simulink library "Steer_Rack_WheelDrivenRack"  (R2025a)
settings: Solver=VariableStepAuto  StartTime=0.0  StopTime=10.0  RelTol=1e-3
undefined symbols (not defined in the file): Steer, Vehicle, Visual, X, Y, Z
libraries: sm_lib x30, nesl_utility x4, Vehicle_Inputs x1, Driver_Systems x1, SteeringWheel x1
Description:
  | Component of Simscape Vehicle Templates Library
  | 
  | Copyright 2018-2026 The MathWorks, Inc.
settings Model: Creator=smiller  LastModifiedBy=smiller
settings OptimizationCC: ReuseModelBlockBuffer=off
settings ModelReferenceCC: EnableRefExpFcnMdlSchedulingChecks=on
settings RTWCC: GPUComputeCapability=3.5

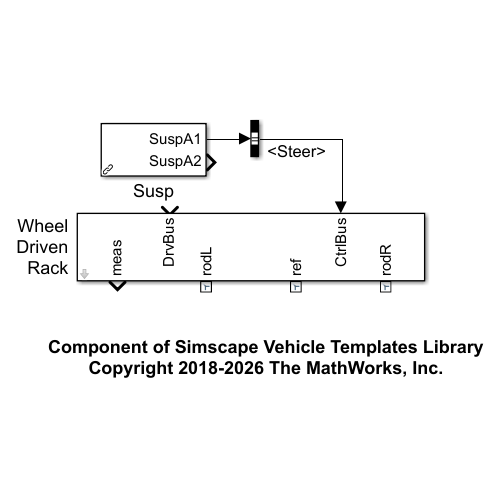
[thumbnail: Simulink's stored preview of the top-level diagram]
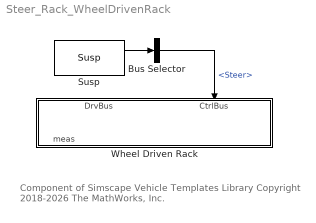
== system Steer_Rack_WheelDrivenRack ==
  note: Component of Simscape Vehicle Templates Library
      | Copyright 2018-2026 The MathWorks, Inc.
  Bus Selector : BusSelector  OutputSignals=Steer
  Susp : Vehicle_Inputs/Control Bus/Susp  SystemSampleTime=-1  VariantActivationTime=update diagram  EmptyChoice=off  PassThrough=off  PassThroughVariantControl=(default)  EmptyChoiceVariantControl=(default)  AllowFlexibleInterface=on  Latency=0  AutoFrameSizeCalculation=off
  Wheel Driven Rack : Subsystem  Tag=PublishSubsystem  VariantControl=Rack  mask(Steering System with Wheel Actuation){hp_wheel=Vehicle.Chassis.SuspF.Steer.Wheel.sMount.Value, wheel_axis_incl=Vehicle.Chassis.SuspF.Steer.Wheel.aAxis.Value, hp_mt_rack=Vehicle.Chassis.SuspF.Steer.Rack.sMount.Value, hp_out_rack=Vehicle.Chassis.SuspF.Steer.Rack.sOutboard.Value, hp_pinion=Vehicle.Chassis.SuspF.Steer.Pinion.sMount.Value, Wheel=Steer.Wheel, len_sha_u=Vehicle.Chassis.SuspF.Steer.Shaft_Upper.xLength.Value, sha_u_mass=Vehicle.Chassis.SuspF.Steer.Shaft_Upper.m.Value, sha_i_mass=Vehicle.Chassis.SuspF.Steer.Shaft_Intermediate.m.Value, len_sha_l=Vehicle.Chassis.SuspF.Steer.Shaft_Lower.xLength.Value, sha_l_mass=Vehicle.Chassis.SuspF.Steer.Shaft_Lower.m.Value, rad_pinion=Vehicle.Chassis.SuspF.Steer.Pinion.xRad.Value, pinion_mass=Vehicle.Chassis.SuspF.Steer.Pinion.m.Value, rack_mass=Vehicle.Chassis.SuspF.Steer.Rack.m.Value, whl2steer_filter=1/Vehicle.Chassis.SuspF.Steer.Rack.fActuatorCutoff.Value, clr_rack=Visual.SteeringRack.clr, opc_rack=Visual.part.opc, radius_rack=Visual.SteeringRack.rad, clr_shaft=Visual.SteeringShafts.clr, opc_shaft=Visual.part.opc, size_shaft=Visual.SteeringShafts.rad, clr_pinion=Visual.SteeringPinion.clr, opc_pinion=Visual.part.opc, len_pinion=Visual.SteeringPinion.len, clr_connhp=Visual.hp.clr, opc_connhp=Visual.hp.opc, size_connhp=Visual.hp.rad, clr_wheel=Visual.SteeringWheel.clr, opc_wheel=Visual.part.opc, DriverHuman=Steer.DriverHuman}
      mask prompts: hp_wheel "HP Wheel [xyz] (m)"; wheel_axis_incl "Wheel Axis Angle (rad)"; hp_mt_rack "HP Rack Mount [xyz] (m)"; hp_out_rack "HP Track Rod Inboard [xyz] (m)"; hp_pinion "HP Pinion [xyz] (m)"; whl2steer_filter "Steer Motion Filter (sec)"; DriverHuman "Driver Human (structure)"
      mask help: Actuation is applied to steering wheel and transmitted to rack via shafts in steering column. Assumes constant gear ratio between pinion and rack.
      mask init:
      | % Calculate inclination of pinion gear about rack travel axis
      | pinion_incl = atan2(hp_mt_rack(1)-hp_pinion(1),hp_mt_rack(3)-hp_pinion(3));
      | 
      | % Calculate endpoints of lower column and upper column
      | hp_col_lower = hp_pinion + [-len_sha_l*cos(pinion_incl) 0 len_sha_l*sin(pinion_incl)];
      | hp_col_upper = hp_wheel  + [+len_sha_u*cos(wheel_axis_incl)  0 -len_sha_u*sin(wheel_axis_incl)];
      | 
      | % Calculate length of intermediate shaft
      | len_sha_int  = norm(hp_col_upper-hp_col_lower);
      mask TypeOptions hp_wheel:
      | Ref to Wheel/Transform
      | HP Wheel/TranslationCartesianOffset
      mask TypeOptions hp_mt_rack:
      | Ref to Rack/Transform
      | HP Rack/TranslationCartesianOffset
      mask TypeOptions hp_out_rack: Rack/hp_out
      mask TypeOptions rack_mass: Rack/rack_mass
      mask TypeOptions whl2steer_filter: Physical Signal/InputFilterTimeConstant
      mask TypeOptions clr_rack: Rack/clr_rack
      mask TypeOptions opc_rack: Rack/opc_rack
      mask TypeOptions radius_rack: Rack/radius_rack
      mask TypeOptions clr_shaft:
      | Shaft
      | Steering/Shaft/GraphicDiffuseColor | Shaft
      | Lower/Shaft/GraphicDiffuseColor | Shaft
      | Intermediate/Shaft/GraphicDiffuseColor
      mask TypeOptions opc_shaft:
      | Shaft
      | Steering/Shaft/GraphicOpacity | Shaft
      | Lower/Shaft/GraphicOpacity | Shaft
      | Intermediate/Shaft/GraphicOpacity
      mask TypeOptions size_shaft:
      | Shaft
      | Steering/Shaft/CylinderRadius | Shaft
      | Lower/Shaft/CylinderRadius | Shaft
      | Intermediate/Shaft/CylinderRadius
      mask TypeOptions clr_pinion: Pinion/Pinion/GraphicDiffuseColor
      mask TypeOptions opc_pinion: Pinion/Pinion/GraphicOpacity
      mask TypeOptions len_pinion: Pinion/Pinion/CylinderLength
      mask TypeOptions clr_connhp:
      | Ref to Rack/Vis
      | Rack
      | Housing/GraphicDiffuseColor | HPs/HP Lower Col/GraphicDiffuseColor | HPs/HP Pinion/GraphicDiffuseColor | HPs/HP Upper Col/GraphicDiffuseColor
      mask TypeOptions opc_connhp:
      | Ref to Rack/Vis
      | Rack
      | Housing/GraphicOpacity | HPs/HP Lower Col/GraphicOpacity | HPs/HP Pinion/GraphicOpacity | HPs/HP Upper Col/GraphicOpacity
      mask TypeOptions size_connhp:
      | Ref to Rack/Vis
      | Rack
      | Housing/SphereRadius | HPs/HP Lower Col/SphereRadius | HPs/HP Pinion/SphereRadius | HPs/HP Upper Col/SphereRadius
      mask TypeOptions clr_wheel: Wheel/clr_wheel
      mask TypeOptions opc_wheel: Wheel/opc_wheel
      mask DialogControl cont_steer Prompt: Steer
      mask DialogControl grp_strparts Prompt: Parts
      mask DialogControl text_strparts_len Prompt: Length/Radius (m)
      mask DialogControl text_strparts_mass Prompt: Mass (kg)
      mask DialogControl text_strparts_wheel Prompt: Wheel
      mask DialogControl text_strparts_wheel_m Prompt: <CAD file>
      mask DialogControl text_strparts_sha_u Prompt: Upper Shaft
      mask DialogControl text_strparts_sha_i Prompt: Intermediate Shaft
      mask DialogControl text_strparts_sha_i_len Prompt: <length upper, lower>
      mask DialogControl text_strparts_sha_len Prompt: Lower Shaft
      mask DialogControl text_strparts_pinion Prompt: Pinion
      mask DialogControl text_strparts_rack Prompt: Rack
      mask DialogControl text_strparts_rack_len Prompt: <HP Rod Inboard>
      mask DialogControl grp_steering Prompt: Steering Input
      mask DialogControl cont_vis_steer Prompt: Visualization
      mask DialogControl text_steer_vis_clr Prompt: Color [RGB]
      mask DialogControl text_steer_vis_opc Prompt: Opac. (0-1)
      mask DialogControl text_steer_vis_size Prompt: Size (m)
      mask DialogControl text_steer_vis_rack Prompt: Rack
      mask DialogControl text_steer_vis_shafts Prompt: Shafts
      mask DialogControl text_steer_vis_pinion Prompt: Pinion
      mask DialogControl text_steer_vis_connhp Prompt: Connections, HP
      mask DialogControl text_steer_vis_wheel Prompt: Wheel
      mask DialogControl text_steer_size_wheel Prompt: <CAD File>
      mask DialogControl cont_driver_human Prompt: Driver Human
  wires:
  Bus Selector/1 -> Wheel Driven Rack/2(CtrlBus)  "<Steer>"
  Susp/1 -> Bus Selector/1

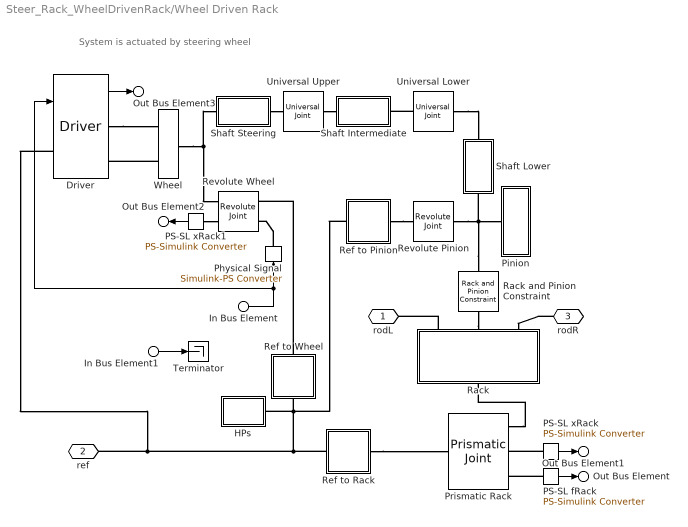
== system Steer_Rack_WheelDrivenRack/Wheel Driven Rack ==
  note: System is actuated by
      | steering wheel
  In Bus Element1 : Inport  PortName=DrvBus  Element=aSteerWheel
  In Bus Element : Inport  Port=2  PortName=CtrlBus  Element=aSteerWheel
  Driver : Driver_Systems/Driver  LabelModeActiveChoice=Human  DriverHuman=DriverHuman  VariantLabel=DriverHuman.class.Value
      settings: AttributesFormatString=%<LabelModeActiveChoice>
  HPs : Subsystem
  PS-SL fRack : nesl_utility/PS-Simulink Converter  PhysicalDomain=network_engine_domain  SubClassName=ps_output  LeftPortType=input  RightPortType=output  PseudoPeriodic=off  Frequencies=[]  VectorFormat=1-D array  Unit=1  AffineConversion=off
  PS-SL xRack : nesl_utility/PS-Simulink Converter  PhysicalDomain=network_engine_domain  SubClassName=ps_output  LeftPortType=input  RightPortType=output  PseudoPeriodic=off  Frequencies=[]  VectorFormat=1-D array  Unit=1  AffineConversion=off
  PS-SL xRack1 : nesl_utility/PS-Simulink Converter  PhysicalDomain=network_engine_domain  SubClassName=ps_output  LeftPortType=input  RightPortType=output  PseudoPeriodic=off  Frequencies=[]  VectorFormat=1-D array  Unit=rad  AffineConversion=off
  Physical Signal : nesl_utility/Simulink-PS Converter  PhysicalDomain=network_engine_domain  SubClassName=ps_input  LeftPortType=input  RightPortType=output  PseudoPeriodic=off  Frequencies=[]  NoiseDistribution=none  NoiseParameters=[]  Unit=rad  AffineConversion=off  FilteringAndDerivatives=filter  SimscapeFilterOrder=2  InputFilterTimeConstant=whl2steer_filter  UdotUserProvided=0
      settings: AttributesFormatString=|
      | Filter Time Constant
      | %<InputFilterTimeConstant> sec
  Pinion : Subsystem
  Prismatic Rack : sm_lib/Joints/Prismatic Joint  JointMode=Normal  CompositeWrenchDir=FollowerOnBase  CompositeWrenchFrame=BaseFrame  SenseConstraintForce=off  SenseConstraintTorque=off  SenseTotalForce=off  SenseTotalTorque=off  PositionTargetSpecify=on  PositionTargetPriority=High  PositionTargetValue=0  PositionTargetValueUnits=m  VelocityTargetSpecify=off  VelocityTargetPriority=High  VelocityTargetValue=0  VelocityTargetValueUnits=m/s  EquilibriumPosition=0  EquilibriumPositionUnits=m  SpringStiffness=0  SpringStiffnessUnits=N/m  DampingCoefficient=1e5*0  DampingCoefficientUnits=N/(m/s)  LowerLimitSpecify=off  LowerLimitBound=-1  LowerLimitBoundUnits=m  LowerLimitStiffness=1e6  LowerLimitStiffnessUnits=N/m  LowerLimitDamping=1e3  LowerLimitDampingUnits=N/(m/s)  LowerLimitTransitionRegionWidth=1e-4  LowerLimitTransitionRegionWidthUnits=m  UpperLimitSpecify=off  UpperLimitBound=1  UpperLimitBoundUnits=m  UpperLimitStiffness=1e6  UpperLimitStiffnessUnits=N/m  UpperLimitDamping=1e3  UpperLimitDampingUnits=N/(m/s)  UpperLimitTransitionRegionWidth=1e-4  UpperLimitTransitionRegionWidthUnits=m  TorqueActuationMode=NoTorque  MotionActuationMode=ComputedMotion  SensePosition=on  SenseVelocity=off  SenseAcceleration=off  SenseTorqueForce=on  SenseLowerLimitTorqueForce=off  SenseUpperLimitTorqueForce=off
  Rack : Subsystem  mask{hp_out=hp_out_rack, rack_mass=rack_mass, clr_rack=clr_rack, opc_rack=opc_rack, radius_rack=radius_rack}
      mask prompts: hp_out "HP Track Rod Inboard [xyz] (m)"; rack_mass "Mass (kg)"
      mask init:
      | rack_length = norm(hp_out-hp_out.*[1 -1 1]);
      mask TypeOptions rack_mass: Rack/Mass
      mask TypeOptions clr_rack: Rack/GraphicDiffuseColor
      mask TypeOptions opc_rack: Rack/GraphicOpacity
      mask TypeOptions radius_rack: Rack/CylinderRadius
      mask DialogControl cont_rack Prompt: Rack
      mask DialogControl text_rack_clr Prompt: Color [RGB]
      mask DialogControl text_rack_opc Prompt: Opac. (0-1)
      mask DialogControl text_rack_size Prompt: Size (m)
      mask DialogControl text_rack_rack Prompt: Rack
  Rack and Pinion Constraint : sm_lib/Gears and Couplings/Gears/Rack and Pinion Constraint  PinionRadius=rad_pinion  PinionRadiusUnits=m
  Ref to Pinion : Subsystem
  Ref to Rack : Subsystem
  Ref to Wheel : Subsystem
  Revolute Pinion : sm_lib/Joints/Revolute Joint  JointMode=Normal  CompositeWrenchDir=FollowerOnBase  CompositeWrenchFrame=BaseFrame  SenseConstraintForce=off  SenseConstraintTorque=off  SenseTotalForce=off  SenseTotalTorque=off  PositionTargetSpecify=off  PositionTargetPriority=High  PositionTargetValue=0  PositionTargetValueUnits=deg  VelocityTargetSpecify=off  VelocityTargetPriority=High  VelocityTargetValue=0  VelocityTargetValueUnits=deg/s  EquilibriumPosition=0  EquilibriumPositionUnits=deg  SpringStiffness=0  SpringStiffnessUnits=N*m/deg  DampingCoefficient=0  DampingCoefficientUnits=N*m/(deg/s)  LowerLimitSpecify=off  LowerLimitBound=-90  LowerLimitBoundUnits=deg  LowerLimitStiffness=1e4  LowerLimitStiffnessUnits=N*m/deg  LowerLimitDamping=10  LowerLimitDampingUnits=N*m/(deg/s)  LowerLimitTransitionRegionWidth=0.1  LowerLimitTransitionRegionWidthUnits=deg  UpperLimitSpecify=off  UpperLimitBound=90  UpperLimitBoundUnits=deg  UpperLimitStiffness=1e4  UpperLimitStiffnessUnits=N*m/deg  UpperLimitDamping=10  UpperLimitDampingUnits=N*m/(deg/s)  UpperLimitTransitionRegionWidth=0.1  UpperLimitTransitionRegionWidthUnits=deg  TorqueActuationMode=NoTorque  MotionActuationMode=ComputedMotion  SensePosition=off  SenseVelocity=off  SenseAcceleration=off  SenseTorqueForce=off  SenseLowerLimitTorqueForce=off  SenseUpperLimitTorqueForce=off
  Revolute Wheel : sm_lib/Joints/Revolute Joint  JointMode=Normal  CompositeWrenchDir=FollowerOnBase  CompositeWrenchFrame=BaseFrame  SenseConstraintForce=off  SenseConstraintTorque=off  SenseTotalForce=off  SenseTotalTorque=off  PositionTargetSpecify=on  PositionTargetPriority=Low  PositionTargetValue=0  PositionTargetValueUnits=deg  VelocityTargetSpecify=off  VelocityTargetPriority=High  VelocityTargetValue=0  VelocityTargetValueUnits=deg/s  EquilibriumPosition=0  EquilibriumPositionUnits=deg  SpringStiffness=0  SpringStiffnessUnits=N*m/deg  DampingCoefficient=0  DampingCoefficientUnits=N*m/(deg/s)  LowerLimitSpecify=off  LowerLimitBound=-90  LowerLimitBoundUnits=deg  LowerLimitStiffness=1e4  LowerLimitStiffnessUnits=N*m/deg  LowerLimitDamping=10  LowerLimitDampingUnits=N*m/(deg/s)  LowerLimitTransitionRegionWidth=0.1  LowerLimitTransitionRegionWidthUnits=deg  UpperLimitSpecify=off  UpperLimitBound=90  UpperLimitBoundUnits=deg  UpperLimitStiffness=1e4  UpperLimitStiffnessUnits=N*m/deg  UpperLimitDamping=10  UpperLimitDampingUnits=N*m/(deg/s)  UpperLimitTransitionRegionWidth=0.1  UpperLimitTransitionRegionWidthUnits=deg  TorqueActuationMode=ComputedTorque  MotionActuationMode=InputMotion  SensePosition=on  SenseVelocity=off  SenseAcceleration=off  SenseTorqueForce=off  SenseLowerLimitTorqueForce=off  SenseUpperLimitTorqueForce=off
  Shaft Intermediate : Subsystem
  Shaft Lower : Subsystem
  Shaft Steering : Subsystem
  Terminator : Terminator
  Universal Lower : sm_lib/Joints/Universal Joint  JointMode=Normal  CompositeWrenchDir=FollowerOnBase  CompositeWrenchFrame=BaseFrame  SenseConstraintForce=off  SenseConstraintTorque=off  SenseTotalForce=off  SenseTotalTorque=off  RxPositionTargetSpecify=off  RxPositionTargetPriority=High  RxPositionTargetValue=0  RxPositionTargetValueUnits=deg  RxVelocityTargetSpecify=off  RxVelocityTargetPriority=High  RxVelocityTargetValue=0  RxVelocityTargetValueUnits=deg/s  RxEquilibriumPosition=0  RxEquilibriumPositionUnits=deg  RxSpringStiffness=0  RxSpringStiffnessUnits=N*m/deg  RxDampingCoefficient=0  RxDampingCoefficientUnits=N*m/(deg/s)  RxLowerLimitSpecify=off  RxLowerLimitBound=-90  RxLowerLimitBoundUnits=deg  RxLowerLimitStiffness=1e4  RxLowerLimitStiffnessUnits=N*m/deg  RxLowerLimitDamping=10  RxLowerLimitDampingUnits=N*m/(deg/s)  RxLowerLimitTransitionRegionWidth=0.1  RxLowerLimitTransitionRegionWidthUnits=deg  RxUpperLimitSpecify=off  RxUpperLimitBound=90  RxUpperLimitBoundUnits=deg  RxUpperLimitStiffness=1e4  RxUpperLimitStiffnessUnits=N*m/deg  RxUpperLimitDamping=10  RxUpperLimitDampingUnits=N*m/(deg/s)  RxUpperLimitTransitionRegionWidth=0.1  RxUpperLimitTransitionRegionWidthUnits=deg  RxTorqueActuationMode=NoTorque  RxMotionActuationMode=ComputedMotion  RxSensePosition=off  RxSenseVelocity=off  RxSenseAcceleration=off  RxSenseTorqueForce=off  RxSenseLowerLimitTorqueForce=off  RxSenseUpperLimitTorqueForce=off  RyPositionTargetSpecify=off  RyPositionTargetPriority=High  RyPositionTargetValue=0  RyPositionTargetValueUnits=deg  RyVelocityTargetSpecify=off  RyVelocityTargetPriority=High  RyVelocityTargetValue=0  RyVelocityTargetValueUnits=deg/s  RyEquilibriumPosition=0  RyEquilibriumPositionUnits=deg  RySpringStiffness=0  RySpringStiffnessUnits=N*m/deg  RyDampingCoefficient=0  RyDampingCoefficientUnits=N*m/(deg/s)  RyLowerLimitSpecify=off  RyLowerLimitBound=-90  RyLowerLimitBoundUnits=deg  RyLowerLimitStiffness=1e4  RyLowerLimitStiffnessUnits=N*m/deg  RyLowerLimitDamping=10  RyLowerLimitDampingUnits=N*m/(deg/s)  RyLowerLimitTransitionRegionWidth=0.1  RyLowerLimitTransitionRegionWidthUnits=deg  RyUpperLimitSpecify=off  RyUpperLimitBound=90  RyUpperLimitBoundUnits=deg  RyUpperLimitStiffness=1e4  RyUpperLimitStiffnessUnits=N*m/deg  RyUpperLimitDamping=10  RyUpperLimitDampingUnits=N*m/(deg/s)  RyUpperLimitTransitionRegionWidth=0.1  RyUpperLimitTransitionRegionWidthUnits=deg  RyTorqueActuationMode=NoTorque  RyMotionActuationMode=ComputedMotion  RySensePosition=off  RySenseVelocity=off  RySenseAcceleration=off  RySenseTorqueForce=off  RySenseLowerLimitTorqueForce=off  RySenseUpperLimitTorqueForce=off
  Universal Upper : sm_lib/Joints/Universal Joint  JointMode=Normal  CompositeWrenchDir=FollowerOnBase  CompositeWrenchFrame=BaseFrame  SenseConstraintForce=off  SenseConstraintTorque=off  SenseTotalForce=off  SenseTotalTorque=off  RxPositionTargetSpecify=off  RxPositionTargetPriority=High  RxPositionTargetValue=0  RxPositionTargetValueUnits=deg  RxVelocityTargetSpecify=off  RxVelocityTargetPriority=High  RxVelocityTargetValue=0  RxVelocityTargetValueUnits=deg/s  RxEquilibriumPosition=0  RxEquilibriumPositionUnits=deg  RxSpringStiffness=0  RxSpringStiffnessUnits=N*m/deg  RxDampingCoefficient=0  RxDampingCoefficientUnits=N*m/(deg/s)  RxLowerLimitSpecify=off  RxLowerLimitBound=-90  RxLowerLimitBoundUnits=deg  RxLowerLimitStiffness=1e4  RxLowerLimitStiffnessUnits=N*m/deg  RxLowerLimitDamping=10  RxLowerLimitDampingUnits=N*m/(deg/s)  RxLowerLimitTransitionRegionWidth=0.1  RxLowerLimitTransitionRegionWidthUnits=deg  RxUpperLimitSpecify=off  RxUpperLimitBound=90  RxUpperLimitBoundUnits=deg  RxUpperLimitStiffness=1e4  RxUpperLimitStiffnessUnits=N*m/deg  RxUpperLimitDamping=10  RxUpperLimitDampingUnits=N*m/(deg/s)  RxUpperLimitTransitionRegionWidth=0.1  RxUpperLimitTransitionRegionWidthUnits=deg  RxTorqueActuationMode=NoTorque  RxMotionActuationMode=ComputedMotion  RxSensePosition=off  RxSenseVelocity=off  RxSenseAcceleration=off  RxSenseTorqueForce=off  RxSenseLowerLimitTorqueForce=off  RxSenseUpperLimitTorqueForce=off  RyPositionTargetSpecify=off  RyPositionTargetPriority=High  RyPositionTargetValue=0  RyPositionTargetValueUnits=deg  RyVelocityTargetSpecify=off  RyVelocityTargetPriority=High  RyVelocityTargetValue=0  RyVelocityTargetValueUnits=deg/s  RyEquilibriumPosition=0  RyEquilibriumPositionUnits=deg  RySpringStiffness=0  RySpringStiffnessUnits=N*m/deg  RyDampingCoefficient=0  RyDampingCoefficientUnits=N*m/(deg/s)  RyLowerLimitSpecify=off  RyLowerLimitBound=-90  RyLowerLimitBoundUnits=deg  RyLowerLimitStiffness=1e4  RyLowerLimitStiffnessUnits=N*m/deg  RyLowerLimitDamping=10  RyLowerLimitDampingUnits=N*m/(deg/s)  RyLowerLimitTransitionRegionWidth=0.1  RyLowerLimitTransitionRegionWidthUnits=deg  RyUpperLimitSpecify=off  RyUpperLimitBound=90  RyUpperLimitBoundUnits=deg  RyUpperLimitStiffness=1e4  RyUpperLimitStiffnessUnits=N*m/deg  RyUpperLimitDamping=10  RyUpperLimitDampingUnits=N*m/(deg/s)  RyUpperLimitTransitionRegionWidth=0.1  RyUpperLimitTransitionRegionWidthUnits=deg  RyTorqueActuationMode=NoTorque  RyMotionActuationMode=ComputedMotion  RySensePosition=off  RySenseVelocity=off  RySenseAcceleration=off  RySenseTorqueForce=off  RySenseLowerLimitTorqueForce=off  RySenseUpperLimitTorqueForce=off
  Wheel : SteeringWheel/Wheel  LabelModeActiveChoice=Sedan  VariantLabel=Wheel.class.Value
  rodL : PMIOPort  Side=Right
  ref : PMIOPort  Port=2  Side=Right
  rodR : PMIOPort  Port=3  Side=Right
  Out Bus Element : Outport  VectorParamsAs1DForOutWhenUnconnected=off  PortName=meas  Element=FRack
  Out Bus Element1 : Outport  VectorParamsAs1DForOutWhenUnconnected=off  PortName=meas  Element=xRack
  Out Bus Element2 : Outport  VectorParamsAs1DForOutWhenUnconnected=off  PortName=meas  Element=aWheel
  Out Bus Element3 : Outport  VectorParamsAs1DForOutWhenUnconnected=off  PortName=meas  Element=Driver
  wires:
  In Bus Element1/1 -> Terminator/1
  Driver/1 -> Out Bus Element3/1
  In Bus Element/1 -> Physical Signal/1, Driver/1
  PS-SL xRack1/1 -> Out Bus Element2/1
  PS-SL xRack/1 -> Out Bus Element1/1
  PS-SL fRack/1 -> Out Bus Element/1
  connections:
  Wheel/RConn2 -- Driver/RConn2
  Driver/RConn1 -- Wheel/RConn1
  Rack and Pinion Constraint/LConn1 -- Shaft Lower/RConn1 -- Pinion/RConn1 -- Revolute Pinion/RConn1
  rodR/RConn1 -- Rack/LConn3
  PS-SL xRack1/LConn1 -- Revolute Wheel/RConn2
  Universal Lower/RConn1 -- Shaft Intermediate/RConn1
  Revolute Wheel/RConn1 -- Shaft Steering/RConn1 -- Wheel/LConn1
  Universal Upper/LConn1 -- Shaft Intermediate/LConn1
  Shaft Steering/LConn1 -- Universal Upper/RConn1
  Universal Lower/LConn1 -- Shaft Lower/LConn1
  Ref to Rack/RConn1 -- Prismatic Rack/LConn1
  Ref to Pinion/RConn1 -- Revolute Pinion/LConn1
  Ref to Wheel/RConn1 -- Revolute Wheel/LConn1
  PS-SL fRack/LConn1 -- Prismatic Rack/RConn3
  Rack/LConn1 -- rodL/RConn1
  HPs/LConn1 -- Ref to Pinion/LConn1 -- Ref to Wheel/LConn1 -- Ref to Rack/LConn1 -- ref/RConn1 -- Driver/LConn1
  PS-SL xRack/LConn1 -- Prismatic Rack/RConn2
  Rack and Pinion Constraint/RConn1 -- Rack/LConn2
  Physical Signal/RConn1 -- Revolute Wheel/LConn2
  Prismatic Rack/RConn1 -- Rack/RConn1

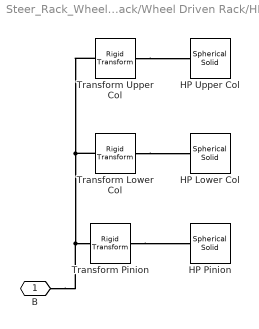
== system Steer_Rack_WheelDrivenRack/Wheel Driven Rack/HPs ==
  HP Lower Col : sm_lib/Body Elements/Spherical Solid  SphereRadius=size_connhp  SphereRadiusUnits=m  ExportEntireGeometry=off  InertiaType=CalculateFromGeometry  BasedOnType=Density  Density=1000  DensityUnits=kg/m^3  Mass=1  MassUnits=kg  CenterOfMass=[0 0 0]  CenterOfMassUnits=m  MomentsOfInertia=[1 1 1]  MomentsOfInertiaUnits=kg*m^2  ProductsOfInertia=[0 0 0]  ProductsOfInertiaUnits=kg*m^2  GraphicType=FromGeometry  MarkerShape=Sphere  MarkerSize=10  GraphicVisPropType=SimpleVisualProperties  GraphicDiffuseColor=clr_connhp  GraphicOpacity=opc_connhp  GraphicSpecularColor=[0.5 0.5 0.5 1.0]  GraphicAmbientColor=[0.15 0.15 0.15 1.0]  GraphicEmissiveColor=[0.0 0.0 0.0 1.0]  GraphicShininess=75  DoExposeReferenceFrame=on  SerializedFrames=<Frames/>
  HP Pinion : sm_lib/Body Elements/Spherical Solid  SphereRadius=size_connhp  SphereRadiusUnits=m  ExportEntireGeometry=off  InertiaType=CalculateFromGeometry  BasedOnType=Density  Density=1000  DensityUnits=kg/m^3  Mass=1  MassUnits=kg  CenterOfMass=[0 0 0]  CenterOfMassUnits=m  MomentsOfInertia=[1 1 1]  MomentsOfInertiaUnits=kg*m^2  ProductsOfInertia=[0 0 0]  ProductsOfInertiaUnits=kg*m^2  GraphicType=FromGeometry  MarkerShape=Sphere  MarkerSize=10  GraphicVisPropType=SimpleVisualProperties  GraphicDiffuseColor=clr_connhp  GraphicOpacity=opc_connhp  GraphicSpecularColor=[0.5 0.5 0.5 1.0]  GraphicAmbientColor=[0.15 0.15 0.15 1.0]  GraphicEmissiveColor=[0.0 0.0 0.0 1.0]  GraphicShininess=75  DoExposeReferenceFrame=on  SerializedFrames=<Frames/>
  HP Upper Col : sm_lib/Body Elements/Spherical Solid  SphereRadius=size_connhp  SphereRadiusUnits=m  ExportEntireGeometry=off  InertiaType=CalculateFromGeometry  BasedOnType=Density  Density=1000  DensityUnits=kg/m^3  Mass=1  MassUnits=kg  CenterOfMass=[0 0 0]  CenterOfMassUnits=m  MomentsOfInertia=[1 1 1]  MomentsOfInertiaUnits=kg*m^2  ProductsOfInertia=[0 0 0]  ProductsOfInertiaUnits=kg*m^2  GraphicType=FromGeometry  MarkerShape=Sphere  MarkerSize=10  GraphicVisPropType=SimpleVisualProperties  GraphicDiffuseColor=clr_connhp  GraphicOpacity=opc_connhp  GraphicSpecularColor=[0.5 0.5 0.5 1.0]  GraphicAmbientColor=[0.15 0.15 0.15 1.0]  GraphicEmissiveColor=[0.0 0.0 0.0 1.0]  GraphicShininess=75  DoExposeReferenceFrame=on  SerializedFrames=<Frames/>
  Transform Lower Col : sm_lib/Frames and Transforms/Rigid Transform  RotationMethod=None  FollAlignAxisA=+X  BaseAlignAxisA=+Y  FollAlignAxisB=+Y  BaseAlignAxisB=+Z  RotationStandardAxis=+Z  RotationAngle=0.0  RotationAngleUnits=deg  RotationArbitraryAxis=[0 0 1]  RotationSequenceAxes=FollowerAxes  RotationSequence=XYX  RotationSequenceAngles=[0 0 0]  RotationSequenceAnglesUnits=deg  RotationMatrix=[1 0 0; 0 1 0; 0 0 1]  Quaternion=[1 0 0 0]  TranslationMethod=Cartesian  TranslationCartesianOffset=hp_col_lower  TranslationCartesianOffsetUnits=m  TranslationStandardAxis=+Z  TranslationStandardOffset=0  TranslationStandardOffsetUnits=m  TranslationROffset=0  TranslationROffsetUnits=m  TranslationThetaOffset=0  TranslationThetaOffsetUnits=deg  TranslationZOffset=0  TranslationZOffsetUnits=m
  Transform Pinion : sm_lib/Frames and Transforms/Rigid Transform  RotationMethod=None  FollAlignAxisA=+X  BaseAlignAxisA=+Y  FollAlignAxisB=+Y  BaseAlignAxisB=+Z  RotationStandardAxis=+Z  RotationAngle=0.0  RotationAngleUnits=deg  RotationArbitraryAxis=[0 0 1]  RotationSequenceAxes=FollowerAxes  RotationSequence=XYX  RotationSequenceAngles=[0 0 0]  RotationSequenceAnglesUnits=deg  RotationMatrix=[1 0 0; 0 1 0; 0 0 1]  Quaternion=[1 0 0 0]  TranslationMethod=Cartesian  TranslationCartesianOffset=hp_pinion  TranslationCartesianOffsetUnits=m  TranslationStandardAxis=+Z  TranslationStandardOffset=0  TranslationStandardOffsetUnits=m  TranslationROffset=0  TranslationROffsetUnits=m  TranslationThetaOffset=0  TranslationThetaOffsetUnits=deg  TranslationZOffset=0  TranslationZOffsetUnits=m
  Transform Upper Col : sm_lib/Frames and Transforms/Rigid Transform  RotationMethod=None  FollAlignAxisA=+X  BaseAlignAxisA=+Y  FollAlignAxisB=+Y  BaseAlignAxisB=+Z  RotationStandardAxis=+Z  RotationAngle=0.0  RotationAngleUnits=deg  RotationArbitraryAxis=[0 0 1]  RotationSequenceAxes=FollowerAxes  RotationSequence=XYX  RotationSequenceAngles=[0 0 0]  RotationSequenceAnglesUnits=deg  RotationMatrix=[1 0 0; 0 1 0; 0 0 1]  Quaternion=[1 0 0 0]  TranslationMethod=Cartesian  TranslationCartesianOffset=hp_col_upper  TranslationCartesianOffsetUnits=m  TranslationStandardAxis=+Z  TranslationStandardOffset=0  TranslationStandardOffsetUnits=m  TranslationROffset=0  TranslationROffsetUnits=m  TranslationThetaOffset=0  TranslationThetaOffsetUnits=deg  TranslationZOffset=0  TranslationZOffsetUnits=m
  B : PMIOPort  Side=Left
  connections:
  Transform Upper Col/RConn1 -- HP Upper Col/RConn1
  Transform Lower Col/RConn1 -- HP Lower Col/RConn1
  Transform Upper Col/LConn1 -- B/RConn1 -- Transform Pinion/LConn1 -- Transform Lower Col/LConn1
  Transform Pinion/RConn1 -- HP Pinion/RConn1

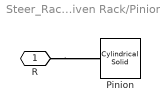
== system Steer_Rack_WheelDrivenRack/Wheel Driven Rack/Pinion ==
  Pinion : sm_lib/Body Elements/Cylindrical Solid  CylinderRadius=rad_pinion  CylinderRadiusUnits=m  CylinderLength=len_pinion  CylinderLengthUnits=m  ExportEntireGeometry=off  InertiaType=CalculateFromGeometry  BasedOnType=Mass  Density=1000  DensityUnits=kg/m^3  Mass=pinion_mass  MassUnits=kg  CenterOfMass=[0 0 0]  CenterOfMassUnits=m  MomentsOfInertia=[1 1 1]  MomentsOfInertiaUnits=kg*m^2  ProductsOfInertia=[0 0 0]  ProductsOfInertiaUnits=kg*m^2  GraphicType=FromGeometry  MarkerShape=Sphere  MarkerSize=10  GraphicVisPropType=SimpleVisualProperties  GraphicDiffuseColor=clr_pinion  GraphicOpacity=opc_pinion  GraphicSpecularColor=[0.5 0.5 0.5 1.0]  GraphicAmbientColor=[0.15 0.15 0.15 1.0]  GraphicEmissiveColor=[0.0 0.0 0.0 1.0]  GraphicShininess=75  DoExposeReferenceFrame=on  SerializedFrames=<Frames/>
  R : PMIOPort  Side=Right
  connections:
  R/RConn1 -- Pinion/RConn1

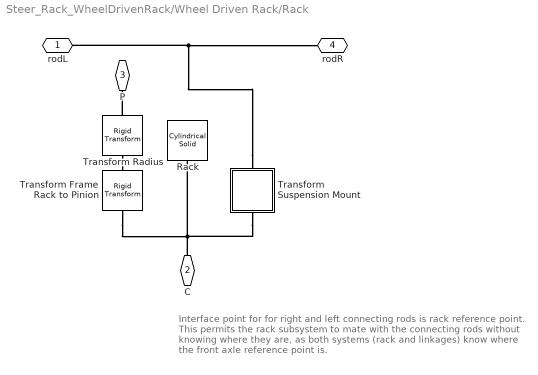
== system Steer_Rack_WheelDrivenRack/Wheel Driven Rack/Rack ==
  note: Interface point for for right and left connecting rods is rack reference point. This permits the rack subsystem to mate with the connecting rods without knowing where they are, as both systems (rack and linkages) know where the front axle reference point is.
  Rack : sm_lib/Body Elements/Cylindrical Solid  CylinderRadius=radius_rack  CylinderRadiusUnits=m  CylinderLength=rack_length  CylinderLengthUnits=m  ExportEntireGeometry=off  InertiaType=CalculateFromGeometry  BasedOnType=Mass  Density=7000  DensityUnits=kg/m^3  Mass=rack_mass  MassUnits=kg  CenterOfMass=[0 0 0]  CenterOfMassUnits=m  MomentsOfInertia=[1 1 1]  MomentsOfInertiaUnits=kg*m^2  ProductsOfInertia=[0 0 0]  ProductsOfInertiaUnits=kg*m^2  GraphicType=FromGeometry  MarkerShape=Sphere  MarkerSize=10  GraphicVisPropType=SimpleVisualProperties  GraphicDiffuseColor=clr_rack  GraphicOpacity=opc_rack  GraphicSpecularColor=[0.5 0.5 0.5 1.0]  GraphicAmbientColor=[0.15 0.15 0.15 1.0]  GraphicEmissiveColor=[0.0 0.0 0.0 1.0]  GraphicShininess=75  DoExposeReferenceFrame=on  SerializedFrames=<Frames/>
  "Transform Frame Rack to Pinion " : sm_lib/Frames and Transforms/Rigid Transform  RotationMethod=StandardAxis  FollAlignAxisA=+X  BaseAlignAxisA=+Y  FollAlignAxisB=+Y  BaseAlignAxisB=+Z  RotationStandardAxis=+Z  RotationAngle=pinion_incl  RotationAngleUnits=rad  RotationArbitraryAxis=[0 0 1]  RotationSequenceAxes=FollowerAxes  RotationSequence=XYX  RotationSequenceAngles=[0 0 0]  RotationSequenceAnglesUnits=deg  RotationMatrix=[1 0 0; 0 1 0; 0 0 1]  Quaternion=[1 0 0 0]  TranslationMethod=StandardAxis  TranslationCartesianOffset=[0 0 0]  TranslationCartesianOffsetUnits=m  TranslationStandardAxis=+Z  TranslationStandardOffset=hp_pinion(2)-hp_mt_rack(2)  TranslationStandardOffsetUnits=m  TranslationROffset=0  TranslationROffsetUnits=m  TranslationThetaOffset=0  TranslationThetaOffsetUnits=deg  TranslationZOffset=0  TranslationZOffsetUnits=m
  Transform Radius : sm_lib/Frames and Transforms/Rigid Transform  RotationMethod=StandardAxis  FollAlignAxisA=+X  BaseAlignAxisA=+Y  FollAlignAxisB=+Y  BaseAlignAxisB=+Z  RotationStandardAxis=+Y  RotationAngle=180  RotationAngleUnits=deg  RotationArbitraryAxis=[0 0 1]  RotationSequenceAxes=FollowerAxes  RotationSequence=XYX  RotationSequenceAngles=[0 0 0]  RotationSequenceAnglesUnits=deg  RotationMatrix=[1 0 0; 0 1 0; 0 0 1]  Quaternion=[1 0 0 0]  TranslationMethod=StandardAxis  TranslationCartesianOffset=[0 0 0]  TranslationCartesianOffsetUnits=m  TranslationStandardAxis=+Y  TranslationStandardOffset=norm(hp_pinion([1 3])-hp_mt_rack([1 3]))-rad_pinion  TranslationStandardOffsetUnits=m  TranslationROffset=0  TranslationROffsetUnits=m  TranslationThetaOffset=0  TranslationThetaOffsetUnits=deg  TranslationZOffset=0  TranslationZOffsetUnits=m
  Transform Suspension Mount : Subsystem
  rodL : PMIOPort  Side=Left
  C : PMIOPort  Port=2  Side=Right
  P : PMIOPort  Port=3  Side=Left
  rodR : PMIOPort  Port=4  Side=Left
  connections:
  Transform Suspension Mount/LConn1 -- rodL/RConn1 -- rodR/RConn1
  Transform Radius/RConn1 -- P/RConn1
  Transform Radius/LConn1 -- "Transform Frame Rack to Pinion "/RConn1
  "Transform Frame Rack to Pinion "/LConn1 -- Transform Suspension Mount/RConn1 -- Rack/RConn1 -- C/RConn1

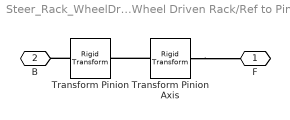
== system Steer_Rack_WheelDrivenRack/Wheel Driven Rack/Ref to Pinion ==
  Transform Pinion : sm_lib/Frames and Transforms/Rigid Transform  RotationMethod=StandardAxis  FollAlignAxisA=+X  BaseAlignAxisA=+Y  FollAlignAxisB=+Y  BaseAlignAxisB=+Z  RotationStandardAxis=+Y  RotationAngle=pinion_incl  RotationAngleUnits=rad  RotationArbitraryAxis=[0 0 1]  RotationSequenceAxes=FollowerAxes  RotationSequence=XYX  RotationSequenceAngles=[0 0 0]  RotationSequenceAnglesUnits=deg  RotationMatrix=[1 0 0; 0 1 0; 0 0 1]  Quaternion=[1 0 0 0]  TranslationMethod=Cartesian  TranslationCartesianOffset=hp_pinion  TranslationCartesianOffsetUnits=m  TranslationStandardAxis=+Z  TranslationStandardOffset=0  TranslationStandardOffsetUnits=m  TranslationROffset=0  TranslationROffsetUnits=m  TranslationThetaOffset=0  TranslationThetaOffsetUnits=deg  TranslationZOffset=0  TranslationZOffsetUnits=m
  Transform Pinion Axis : sm_lib/Frames and Transforms/Rigid Transform  RotationMethod=RotationSequence  FollAlignAxisA=+X  BaseAlignAxisA=+Y  FollAlignAxisB=+Y  BaseAlignAxisB=+Z  RotationStandardAxis=+Y  RotationAngle=0  RotationAngleUnits=rad  RotationArbitraryAxis=[0 0 1]  RotationSequenceAxes=FollowerAxes  RotationSequence=ZXZ  RotationSequenceAngles=[-90 -90 0]  RotationSequenceAnglesUnits=deg  RotationMatrix=[1 0 0; 0 1 0; 0 0 1]  Quaternion=[1 0 0 0]  TranslationMethod=None  TranslationCartesianOffset=[0 0 0]  TranslationCartesianOffsetUnits=m  TranslationStandardAxis=+Z  TranslationStandardOffset=0  TranslationStandardOffsetUnits=m  TranslationROffset=0  TranslationROffsetUnits=m  TranslationThetaOffset=0  TranslationThetaOffsetUnits=deg  TranslationZOffset=0  TranslationZOffsetUnits=m
  F : PMIOPort  Side=Right
  B : PMIOPort  Port=2  Side=Left
  connections:
  Transform Pinion Axis/RConn1 -- F/RConn1
  Transform Pinion/LConn1 -- B/RConn1
  Transform Pinion Axis/LConn1 -- Transform Pinion/RConn1

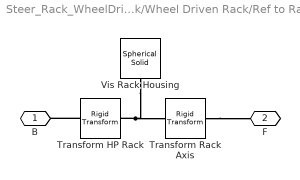
== system Steer_Rack_WheelDrivenRack/Wheel Driven Rack/Ref to Rack ==
  Transform HP Rack : sm_lib/Frames and Transforms/Rigid Transform  RotationMethod=None  FollAlignAxisA=+X  BaseAlignAxisA=+Y  FollAlignAxisB=+Y  BaseAlignAxisB=+Z  RotationStandardAxis=+Z  RotationAngle=0.0  RotationAngleUnits=deg  RotationArbitraryAxis=[0 0 1]  RotationSequenceAxes=FollowerAxes  RotationSequence=XYX  RotationSequenceAngles=[0 0 0]  RotationSequenceAnglesUnits=deg  RotationMatrix=[1 0 0; 0 1 0; 0 0 1]  Quaternion=[1 0 0 0]  TranslationMethod=Cartesian  TranslationCartesianOffset=hp_mt_rack  TranslationCartesianOffsetUnits=m  TranslationStandardAxis=+Z  TranslationStandardOffset=0  TranslationStandardOffsetUnits=m  TranslationROffset=0  TranslationROffsetUnits=m  TranslationThetaOffset=0  TranslationThetaOffsetUnits=deg  TranslationZOffset=0  TranslationZOffsetUnits=m
  Transform Rack Axis : sm_lib/Frames and Transforms/Rigid Transform  RotationMethod=AlignedAxes  FollAlignAxisA=+Y  BaseAlignAxisA=-Z  FollAlignAxisB=+X  BaseAlignAxisB=+X  RotationStandardAxis=+Z  RotationAngle=0  RotationAngleUnits=deg  RotationArbitraryAxis=[0 0 1]  RotationSequenceAxes=FollowerAxes  RotationSequence=XYX  RotationSequenceAngles=[0 0 0]  RotationSequenceAnglesUnits=deg  RotationMatrix=[0 0 -1;0 1 0;1 0 0]  Quaternion=[1 0 0 0]  TranslationMethod=None  TranslationCartesianOffset=[0 0 0]  TranslationCartesianOffsetUnits=m  TranslationStandardAxis=+Z  TranslationStandardOffset=0  TranslationStandardOffsetUnits=m  TranslationROffset=0  TranslationROffsetUnits=m  TranslationThetaOffset=0  TranslationThetaOffsetUnits=deg  TranslationZOffset=0  TranslationZOffsetUnits=m
  Vis Rack Housing : sm_lib/Body Elements/Spherical Solid  SphereRadius=size_connhp  SphereRadiusUnits=m  ExportEntireGeometry=off  InertiaType=CalculateFromGeometry  BasedOnType=Density  Density=1000  DensityUnits=kg/m^3  Mass=1  MassUnits=kg  CenterOfMass=[0 0 0]  CenterOfMassUnits=m  MomentsOfInertia=[1 1 1]  MomentsOfInertiaUnits=kg*m^2  ProductsOfInertia=[0 0 0]  ProductsOfInertiaUnits=kg*m^2  GraphicType=FromGeometry  MarkerShape=Sphere  MarkerSize=10  GraphicVisPropType=SimpleVisualProperties  GraphicDiffuseColor=clr_connhp  GraphicOpacity=opc_connhp  GraphicSpecularColor=[0.5 0.5 0.5 1.0]  GraphicAmbientColor=[0.15 0.15 0.15 1.0]  GraphicEmissiveColor=[0.0 0.0 0.0 1.0]  GraphicShininess=75  DoExposeReferenceFrame=on  SerializedFrames=<Frames/>
  B : PMIOPort  Side=Left
  F : PMIOPort  Port=2  Side=Right
  connections:
  Transform HP Rack/LConn1 -- B/RConn1
  Transform Rack Axis/RConn1 -- F/RConn1
  Transform HP Rack/RConn1 -- Vis Rack Housing/RConn1 -- Transform Rack Axis/LConn1

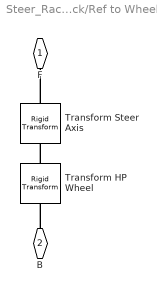
== system Steer_Rack_WheelDrivenRack/Wheel Driven Rack/Ref to Wheel ==
  Transform HP Wheel : sm_lib/Frames and Transforms/Rigid Transform  RotationMethod=None  FollAlignAxisA=+X  BaseAlignAxisA=+Y  FollAlignAxisB=+Y  BaseAlignAxisB=+Z  RotationStandardAxis=+Z  RotationAngle=0.0  RotationAngleUnits=deg  RotationArbitraryAxis=[0 0 1]  RotationSequenceAxes=FollowerAxes  RotationSequence=XYX  RotationSequenceAngles=[0 0 0]  RotationSequenceAnglesUnits=deg  RotationMatrix=[1 0 0; 0 1 0; 0 0 1]  Quaternion=[1 0 0 0]  TranslationMethod=Cartesian  TranslationCartesianOffset=hp_wheel  TranslationCartesianOffsetUnits=m  TranslationStandardAxis=+Z  TranslationStandardOffset=0  TranslationStandardOffsetUnits=m  TranslationROffset=0  TranslationROffsetUnits=m  TranslationThetaOffset=0  TranslationThetaOffsetUnits=deg  TranslationZOffset=0  TranslationZOffsetUnits=m
  Transform Steer Axis : sm_lib/Frames and Transforms/Rigid Transform  RotationMethod=StandardAxis  FollAlignAxisA=+X  BaseAlignAxisA=+Y  FollAlignAxisB=+Y  BaseAlignAxisB=+Z  RotationStandardAxis=+Y  RotationAngle=-pi/2+wheel_axis_incl  RotationAngleUnits=rad  RotationArbitraryAxis=[0 0 1]  RotationSequenceAxes=FollowerAxes  RotationSequence=XYX  RotationSequenceAngles=[0 0 0]  RotationSequenceAnglesUnits=deg  RotationMatrix=[1 0 0; 0 1 0; 0 0 1]  Quaternion=[1 0 0 0]  TranslationMethod=None  TranslationCartesianOffset=[0 0 0]  TranslationCartesianOffsetUnits=m  TranslationStandardAxis=+Z  TranslationStandardOffset=0  TranslationStandardOffsetUnits=m  TranslationROffset=0  TranslationROffsetUnits=m  TranslationThetaOffset=0  TranslationThetaOffsetUnits=deg  TranslationZOffset=0  TranslationZOffsetUnits=m
  F : PMIOPort  Side=Right
  B : PMIOPort  Port=2  Side=Left
  connections:
  Transform Steer Axis/RConn1 -- F/RConn1
  B/RConn1 -- Transform HP Wheel/LConn1
  Transform HP Wheel/RConn1 -- Transform Steer Axis/LConn1

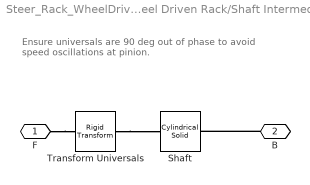
== system Steer_Rack_WheelDrivenRack/Wheel Driven Rack/Shaft Intermediate ==
  note: Ensure universals are 90 deg out of phase to avoid speed oscillations at pinion.
  Shaft : sm_lib/Body Elements/Cylindrical Solid  CylinderRadius=size_shaft  CylinderRadiusUnits=m  CylinderLength=norm(hp_col_lower-hp_col_upper)  CylinderLengthUnits=m  ExportEntireGeometry=off  InertiaType=CalculateFromGeometry  BasedOnType=Mass  Density=1000  DensityUnits=kg/m^3  Mass=sha_i_mass  MassUnits=kg  CenterOfMass=[0 0 0]  CenterOfMassUnits=m  MomentsOfInertia=[1 1 1]  MomentsOfInertiaUnits=kg*m^2  ProductsOfInertia=[0 0 0]  ProductsOfInertiaUnits=kg*m^2  GraphicType=FromGeometry  MarkerShape=Sphere  MarkerSize=10  GraphicVisPropType=SimpleVisualProperties  GraphicDiffuseColor=clr_shaft  GraphicOpacity=opc_shaft  GraphicSpecularColor=[0.5 0.5 0.5 1.0]  GraphicAmbientColor=[0.15 0.15 0.15 1.0]  GraphicEmissiveColor=[0.0 0.0 0.0 1.0]  GraphicShininess=75  DoExposeReferenceFrame=off  SerializedFrames=<Frames><Frame><Id>Frame1</Id><Value><Name>B</Name><Origin><Source>GeometricFeature</Source><FeatureName>bottom surface</FeatureName></Origin><PrimaryAxis><DefinedDirection>+Z</DefinedDirection><Source>ReferenceFrame</Source><SourceDirection>+Z</SourceDirection><FeatureName></FeatureName></PrimaryAxis><SecondaryAxis><DefinedDirection>+X</DefinedDirection><Source>ReferenceFrame</Source><SourceDirection>+X</SourceDirection><FeatureName></FeatureName></SecondaryAxis></Value></Frame><Frame><Id>Frame2</Id><Value><Name>F</Name><Origin><Source>GeometricFeature</Source><FeatureName>top curve</FeatureName></Origin><PrimaryAxis><DefinedDirection>+Z</DefinedDirection><Source>ReferenceFrame</Source><SourceDirection>+Z</SourceDirection><FeatureName></FeatureName></PrimaryAxis><SecondaryAxis><DefinedDirection>+X</DefinedDirection><Source>ReferenceFrame</Source><SourceDirection>+X</SourceDirection><FeatureName></FeatureName></SecondaryAxis></Value></Frame></Frames>
  Transform Universals : sm_lib/Frames and Transforms/Rigid Transform  RotationMethod=StandardAxis  FollAlignAxisA=+X  BaseAlignAxisA=+Y  FollAlignAxisB=+Y  BaseAlignAxisB=+Z  RotationStandardAxis=+Z  RotationAngle=-90  RotationAngleUnits=deg  RotationArbitraryAxis=[0 0 1]  RotationSequenceAxes=FollowerAxes  RotationSequence=XYX  RotationSequenceAngles=[0 0 0]  RotationSequenceAnglesUnits=deg  RotationMatrix=[1 0 0; 0 1 0; 0 0 1]  Quaternion=[1 0 0 0]  TranslationMethod=None  TranslationCartesianOffset=[0 0 0]  TranslationCartesianOffsetUnits=m  TranslationStandardAxis=+Z  TranslationStandardOffset=0  TranslationStandardOffsetUnits=m  TranslationROffset=0  TranslationROffsetUnits=m  TranslationThetaOffset=0  TranslationThetaOffsetUnits=deg  TranslationZOffset=0  TranslationZOffsetUnits=m
  F : PMIOPort  Side=Left
  B : PMIOPort  Port=2  Side=Right
  connections:
  Transform Universals/RConn1 -- Shaft/RConn1
  B/RConn1 -- Shaft/LConn1
  F/RConn1 -- Transform Universals/LConn1

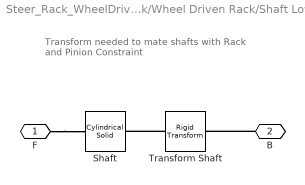
== system Steer_Rack_WheelDrivenRack/Wheel Driven Rack/Shaft Lower ==
  note: Transform needed to mate shafts with Rack and Pinion Constraint
  Shaft : sm_lib/Body Elements/Cylindrical Solid  CylinderRadius=size_shaft  CylinderRadiusUnits=m  CylinderLength=norm(hp_pinion-hp_col_lower)  CylinderLengthUnits=m  ExportEntireGeometry=off  InertiaType=CalculateFromGeometry  BasedOnType=Mass  Density=1000  DensityUnits=kg/m^3  Mass=sha_l_mass  MassUnits=kg  CenterOfMass=[0 0 0]  CenterOfMassUnits=m  MomentsOfInertia=[1 1 1]  MomentsOfInertiaUnits=kg*m^2  ProductsOfInertia=[0 0 0]  ProductsOfInertiaUnits=kg*m^2  GraphicType=FromGeometry  MarkerShape=Sphere  MarkerSize=10  GraphicVisPropType=SimpleVisualProperties  GraphicDiffuseColor=clr_shaft  GraphicOpacity=opc_shaft  GraphicSpecularColor=[0.5 0.5 0.5 1.0]  GraphicAmbientColor=[0.15 0.15 0.15 1.0]  GraphicEmissiveColor=[0.0 0.0 0.0 1.0]  GraphicShininess=75  DoExposeReferenceFrame=off  SerializedFrames=<Frames><Frame><Id>Frame1</Id><Value><Name>B</Name><Origin><Source>GeometricFeature</Source><FeatureName>bottom surface</FeatureName></Origin><PrimaryAxis><DefinedDirection>+Z</DefinedDirection><Source>ReferenceFrame</Source><SourceDirection>+Z</SourceDirection><FeatureName></FeatureName></PrimaryAxis><SecondaryAxis><DefinedDirection>+X</DefinedDirection><Source>ReferenceFrame</Source><SourceDirection>+X</SourceDirection><FeatureName></FeatureName></SecondaryAxis></Value></Frame><Frame><Id>Frame2</Id><Value><Name>F</Name><Origin><Source>GeometricFeature</Source><FeatureName>top curve</FeatureName></Origin><PrimaryAxis><DefinedDirection>+Z</DefinedDirection><Source>ReferenceFrame</Source><SourceDirection>+Z</SourceDirection><FeatureName></FeatureName></PrimaryAxis><SecondaryAxis><DefinedDirection>+X</DefinedDirection><Source>ReferenceFrame</Source><SourceDirection>+X</SourceDirection><FeatureName></FeatureName></SecondaryAxis></Value></Frame></Frames>
  Transform Shaft : sm_lib/Frames and Transforms/Rigid Transform  RotationMethod=StandardAxis  FollAlignAxisA=+X  BaseAlignAxisA=+Y  FollAlignAxisB=+Y  BaseAlignAxisB=+Z  RotationStandardAxis=+X  RotationAngle=180  RotationAngleUnits=deg  RotationArbitraryAxis=[0 0 1]  RotationSequenceAxes=FollowerAxes  RotationSequence=XYX  RotationSequenceAngles=[0 0 0]  RotationSequenceAnglesUnits=deg  RotationMatrix=[1 0 0; 0 1 0; 0 0 1]  Quaternion=[1 0 0 0]  TranslationMethod=None  TranslationCartesianOffset=[0 0 0]  TranslationCartesianOffsetUnits=m  TranslationStandardAxis=+Z  TranslationStandardOffset=0  TranslationStandardOffsetUnits=m  TranslationROffset=0  TranslationROffsetUnits=m  TranslationThetaOffset=0  TranslationThetaOffsetUnits=deg  TranslationZOffset=0  TranslationZOffsetUnits=m
  F : PMIOPort  Side=Left
  B : PMIOPort  Port=2  Side=Right
  connections:
  F/RConn1 -- Shaft/RConn1
  B/RConn1 -- Transform Shaft/LConn1
  Transform Shaft/RConn1 -- Shaft/LConn1

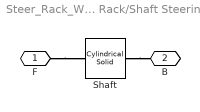
== system Steer_Rack_WheelDrivenRack/Wheel Driven Rack/Shaft Steering ==
  Shaft : sm_lib/Body Elements/Cylindrical Solid  CylinderRadius=size_shaft  CylinderRadiusUnits=m  CylinderLength=norm(hp_col_upper-hp_wheel)  CylinderLengthUnits=m  ExportEntireGeometry=off  InertiaType=CalculateFromGeometry  BasedOnType=Mass  Density=1000  DensityUnits=kg/m^3  Mass=sha_u_mass  MassUnits=kg  CenterOfMass=[0 0 0]  CenterOfMassUnits=m  MomentsOfInertia=[1 1 1]  MomentsOfInertiaUnits=kg*m^2  ProductsOfInertia=[0 0 0]  ProductsOfInertiaUnits=kg*m^2  GraphicType=FromGeometry  MarkerShape=Sphere  MarkerSize=10  GraphicVisPropType=SimpleVisualProperties  GraphicDiffuseColor=clr_shaft  GraphicOpacity=opc_shaft  GraphicSpecularColor=[0.5 0.5 0.5 1.0]  GraphicAmbientColor=[0.15 0.15 0.15 1.0]  GraphicEmissiveColor=[0.0 0.0 0.0 1.0]  GraphicShininess=75  DoExposeReferenceFrame=off  SerializedFrames=<Frames><Frame><Id>Frame1</Id><Value><Name>B</Name><Origin><Source>GeometricFeature</Source><FeatureName>bottom surface</FeatureName></Origin><PrimaryAxis><DefinedDirection>+Z</DefinedDirection><Source>ReferenceFrame</Source><SourceDirection>+Z</SourceDirection><FeatureName></FeatureName></PrimaryAxis><SecondaryAxis><DefinedDirection>+X</DefinedDirection><Source>ReferenceFrame</Source><SourceDirection>+X</SourceDirection><FeatureName></FeatureName></SecondaryAxis></Value></Frame><Frame><Id>Frame2</Id><Value><Name>F</Name><Origin><Source>GeometricFeature</Source><FeatureName>top curve</FeatureName></Origin><PrimaryAxis><DefinedDirection>+Z</DefinedDirection><Source>ReferenceFrame</Source><SourceDirection>+Z</SourceDirection><FeatureName></FeatureName></PrimaryAxis><SecondaryAxis><DefinedDirection>+X</DefinedDirection><Source>ReferenceFrame</Source><SourceDirection>+X</SourceDirection><FeatureName></FeatureName></SecondaryAxis></Value></Frame></Frames>
  F : PMIOPort  Side=Right
  B : PMIOPort  Port=2  Side=Left
  connections:
  F/RConn1 -- Shaft/RConn1
  Shaft/LConn1 -- B/RConn1

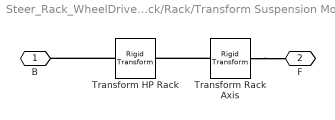
== system Steer_Rack_WheelDrivenRack/Wheel Driven Rack/Rack/Transform Suspension Mount ==
  Transform HP Rack : sm_lib/Frames and Transforms/Rigid Transform  RotationMethod=None  FollAlignAxisA=+X  BaseAlignAxisA=+Y  FollAlignAxisB=+Y  BaseAlignAxisB=+Z  RotationStandardAxis=+Z  RotationAngle=0.0  RotationAngleUnits=deg  RotationArbitraryAxis=[0 0 1]  RotationSequenceAxes=FollowerAxes  RotationSequence=XYX  RotationSequenceAngles=[0 0 0]  RotationSequenceAnglesUnits=deg  RotationMatrix=[1 0 0; 0 1 0; 0 0 1]  Quaternion=[1 0 0 0]  TranslationMethod=Cartesian  TranslationCartesianOffset=hp_mt_rack  TranslationCartesianOffsetUnits=m  TranslationStandardAxis=+Z  TranslationStandardOffset=0  TranslationStandardOffsetUnits=m  TranslationROffset=0  TranslationROffsetUnits=m  TranslationThetaOffset=0  TranslationThetaOffsetUnits=deg  TranslationZOffset=0  TranslationZOffsetUnits=m
  Transform Rack Axis : sm_lib/Frames and Transforms/Rigid Transform  RotationMethod=AlignedAxes  FollAlignAxisA=+Y  BaseAlignAxisA=-Z  FollAlignAxisB=+X  BaseAlignAxisB=+X  RotationStandardAxis=+Z  RotationAngle=0  RotationAngleUnits=deg  RotationArbitraryAxis=[0 0 1]  RotationSequenceAxes=FollowerAxes  RotationSequence=XYX  RotationSequenceAngles=[0 0 0]  RotationSequenceAnglesUnits=deg  RotationMatrix=[0 0 -1;0 1 0;1 0 0]  Quaternion=[1 0 0 0]  TranslationMethod=None  TranslationCartesianOffset=[0 0 0]  TranslationCartesianOffsetUnits=m  TranslationStandardAxis=+Z  TranslationStandardOffset=0  TranslationStandardOffsetUnits=m  TranslationROffset=0  TranslationROffsetUnits=m  TranslationThetaOffset=0  TranslationThetaOffsetUnits=deg  TranslationZOffset=0  TranslationZOffsetUnits=m
  B : PMIOPort  Side=Left
  F : PMIOPort  Port=2  Side=Right
  connections:
  Transform Rack Axis/LConn1 -- Transform HP Rack/RConn1
  Transform HP Rack/LConn1 -- B/RConn1
  Transform Rack Axis/RConn1 -- F/RConn1
